simulink model "fi_at"  (R2026a)
settings: Solver=ode5  StopTime=30  FixedStep=.01  AbsTol=1e-6
model workspace (MATLAB code in the model file):
  | load sldemo_autotrans_data; %load initial conditions and other necessary data
undefined symbols (not defined in the file or in its folder): converter_data, downtab, emap, Iei, uptab, vehicledata
Description:
  | Modeling an Automatic Transmission Controller
  | 
  | In this example, Simulink(R) is used to model an automotive drivetrain. Stateflow(R)
  | enhances the Simulink model with its representation of the transmission
  | control logic. Simulink provides a powerful environment for the modeling and
  | simulation of dynamic systems and processes. In many systems, though,
  | supervisory functions like changing modes or invoking new gain schedules must
  | respond to events that may occur and conditions that develop over time. As a
  | result, the environment requires a language capable of managing these multiple
  | modes and developing conditions. In the following example, Stateflow
  | demonstrates its strength in this capacity by performing the function of gear
  | selection in an automatic transmission. This function is combined with the
  | drivetrain dynamics in a natural and intuitive manner by incorporating a
  | Stateflow block in the Simulink block diagram.
settings Model: DataTypeOverride=Double  MinMaxOverflowLogging=ForceOff  SimulationMode=accelerator  ExtModeTrigMode=oneshot  ExtModeArmWhenConnect=off  ExtModeAutoUpdateStatusClock=off  Creator=The MathWorks Inc.  LastModifiedBy=harry_31916
settings DataIOCC: ExternalInput=[t__, u__]  SignalLoggingName=sldemo_autotrans_output
settings OptimizationCC: BooleanDataType=off  InitFltsAndDblsToZero=on
settings DebuggingCC: SaveWithParameterizedLinksMsg=none  UnderspecifiedInitializationDetection=Classic  CheckExecutionContextPreStartOutputMsg=on  SignalResolutionControl=TryResolveAllWithWarning  MultiTaskDSMMsg=warning  MultiTaskCondExecSysMsg=none  SigSpecEnsureSampleTimeMsg=none  IntegerOverflowMsg=none  IntegerSaturationMsg=none
settings HardwareCC: ProdHWDeviceType=32-bit Generic
settings SFSimCC: SFSimEcho=off
settings GRTTargetCC: TargetFcnLib=ansi_tfl_tmw.mat  CombineOutputUpdateFcns=off  GRTInterface=on
settings ConfigComp: CovMetricSettings=dcmtr

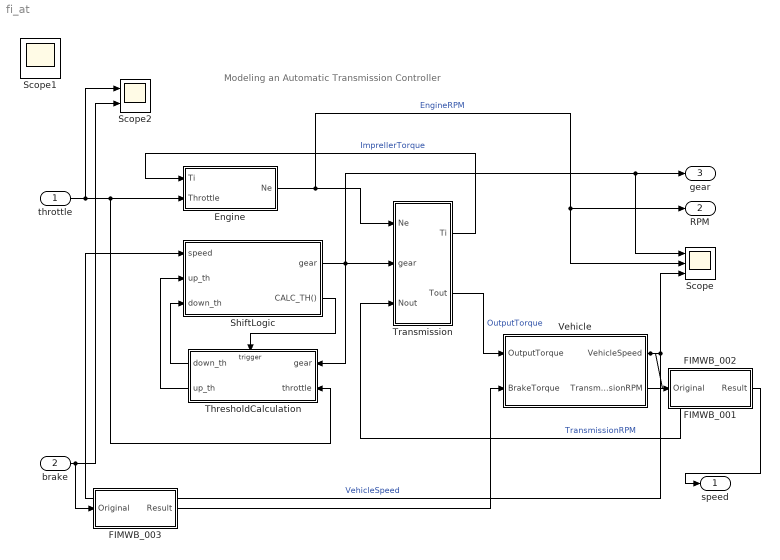
== system fi_at ==
  note: Modeling an Automatic Transmission Controller
  throttle : Inport  Interpolate=off
  brake : Inport  Port=2  Interpolate=off
  Engine : Subsystem
  FIMWB_001 : Subsystem  Tag=fimwb.fault.1
  FIMWB_002 : Subsystem  Tag=fimwb.fault.2
  FIMWB_003 : Subsystem  Tag=fimwb.fault.3
  Scope : Scope  NumInputPorts=3
      settings: ActiveDisplayYMinimum=-5  ActiveDisplayYMaximum=5
  Scope2 : Scope  NumInputPorts=2
      settings: ActiveDisplayYMinimum=-5  ActiveDisplayYMaximum=100
  ShiftLogic : Stateflow chart  TreatAsAtomicUnit=on
  ThresholdCalculation : Subsystem  TreatAsAtomicUnit=on
  Transmission : Subsystem
  Vehicle : Subsystem  mask(vehicle model){Rfd=vehicledata(1), rload0=vehicledata(2), rload2=vehicledata(3), Rw=vehicledata(4), Iv=vehicledata(5), N20=vehicledata(6)/vehicledata(4)*vehicledata(1)}
      mask prompts: Rfd "final drive ratio"; rload0 "drag friction at wheels"; rload2 "aerodynamic drag"; Rw "wheel radius"; Iv "vehicle inertia"; N20 "initial transmission output speed"
      mask help: vehicle dynamics: torque input from trans., outputs are input speed (transmission output) and vehicle speed
      mask Display: image(imread([matlabroot,'/toolbox/simulink/simdemos/automotive/html/NSX_3Colors.jpg']))
  speed : Outport  VectorParamsAs1DForOutWhenUnconnected=off
  RPM : Outport  Port=2  VectorParamsAs1DForOutWhenUnconnected=off
  gear : Outport  Port=3  VectorParamsAs1DForOutWhenUnconnected=off
  Scope1 : Scope
      settings: TimeSpan=30  ActiveDisplayYMinimum=1000  ActiveDisplayYMaximum=5000  DataLoggingMaxPoints=7500  DataLoggingSaveFormat=Array
  wires:
  Transmission/1(Ti) -> Engine/1(Ti)  "ImprellerTorque"
  Engine/1(Ne) -> Transmission/1(Ne), RPM/1, Scope/2  "EngineRPM"
  Vehicle/2(TransmissionRPM) -> Transmission/3(Nout)  "TransmissionRPM"
  ThresholdCalculation/1(down_th) -> ShiftLogic/3(down_th)
  ThresholdCalculation/2(up_th) -> ShiftLogic/2(up_th)
  ShiftLogic/1(gear) -> Transmission/2(gear), ThresholdCalculation/1(gear), gear/1, Scope/1
  ShiftLogic/2(CALC_TH()) -> ThresholdCalculation/Trigger
  Vehicle/1(VehicleSpeed) -> Scope/3, ShiftLogic/1(speed), FIMWB_001/1(Original)  "VehicleSpeed"
  throttle/1 -> Engine/2(Throttle), ThresholdCalculation/2(throttle), Scope2/1
  Transmission/2(Tout) -> Vehicle/1(OutputTorque)  "OutputTorque"
  brake/1 -> Scope2/2, FIMWB_003/1(Original)
  FIMWB_001/1(Result) -> FIMWB_002/1(Original)
  FIMWB_002/1(Result) -> speed/1
  FIMWB_003/1(Result) -> Vehicle/2(BrakeTorque)

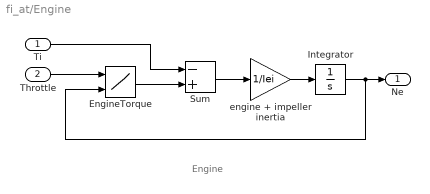
== system fi_at/Engine ==
  note: Engine
  Ti : Inport
  Throttle : Inport  Port=2
  EngineTorque : Lookup2D  RowIndex=thvec  ColumnIndex=nevec  Table=emap  SaturateOnIntegerOverflow=off
  Integrator : Integrator  InitialCondition=1000  LimitOutput=on  UpperSaturationLimit=6000  LowerSaturationLimit=600  ZeroCross=off
  Sum : Sum  Inputs=-+  InputSameDT=on  SaturateOnIntegerOverflow=on  OutDataTypeStr=Inherit: Same as first input
  engine + impeller inertia : Gain  Gain=1/Iei  SaturateOnIntegerOverflow=on  OutDataTypeStr=Inherit: Same as input  ParamDataTypeStr=Inherit: Same as input
  Ne : Outport  InitialOutput=0  VectorParamsAs1DForOutWhenUnconnected=off
  wires:
  Ti/1 -> Sum/1
  Throttle/1 -> EngineTorque/1
  Integrator/1 -> EngineTorque/2, Ne/1
  Sum/1 -> engine + impeller inertia/1
  engine + impeller inertia/1 -> Integrator/1
  EngineTorque/1 -> Sum/2

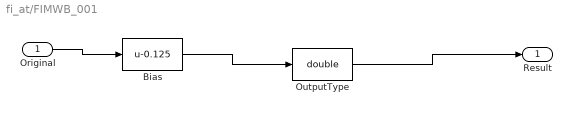
== system fi_at/FIMWB_001 ==
  Original : Inport
  Bias : Bias  Bias=-0.125  SaturateOnIntegerOverflow=off
  OutputType : DataTypeConversion  OutDataTypeStr=double  RndMeth=Round
  Result : Outport
  wires:
  Original/1 -> Bias/1
  Bias/1 -> OutputType/1
  OutputType/1 -> Result/1

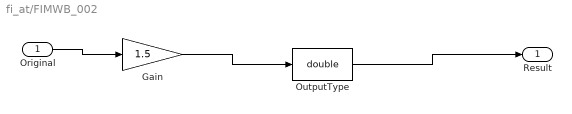
== system fi_at/FIMWB_002 ==
  Original : Inport
  Gain : Gain  Gain=1.5  OutDataTypeStr=Inherit: Same as input
  OutputType : DataTypeConversion  OutDataTypeStr=double  RndMeth=Round
  Result : Outport
  wires:
  Original/1 -> Gain/1
  Gain/1 -> OutputType/1
  OutputType/1 -> Result/1

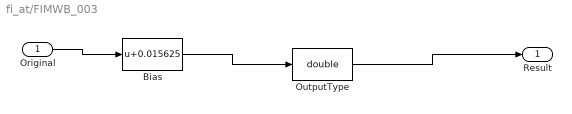
== system fi_at/FIMWB_003 ==
  Original : Inport
  Bias : Bias  Bias=0.015625  SaturateOnIntegerOverflow=off
  OutputType : DataTypeConversion  OutDataTypeStr=double  RndMeth=Round
  Result : Outport
  wires:
  Original/1 -> Bias/1
  Bias/1 -> OutputType/1
  OutputType/1 -> Result/1

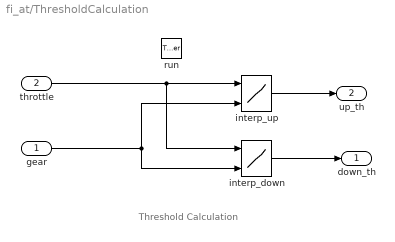
== system fi_at/ThresholdCalculation ==
  note: Threshold Calculation
  gear : Inport
  throttle : Inport  Port=2
  run : TriggerPort  TriggerType=function-call  VariantControl=(inherit)  ZeroCross=off
  interp_down : Lookup2D  RowIndex=downth  ColumnIndex=[1:4]  Table=downtab  OutDataTypeStr=double  SaturateOnIntegerOverflow=off  InputSameDT=off
      settings: LockScale=on
  interp_up : Lookup2D  RowIndex=upth  ColumnIndex=[1:4]  Table=uptab  OutDataTypeStr=double  SaturateOnIntegerOverflow=off  InputSameDT=off
      settings: LockScale=on
  down_th : Outport  VectorParamsAs1DForOutWhenUnconnected=off
  up_th : Outport  Port=2  VectorParamsAs1DForOutWhenUnconnected=off
  wires:
  interp_up/1 -> up_th/1
  interp_down/1 -> down_th/1
  throttle/1 -> interp_up/1, interp_down/1
  gear/1 -> interp_up/2, interp_down/2

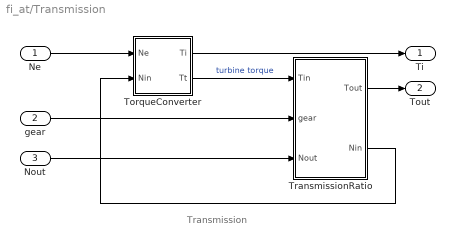
== system fi_at/Transmission ==
  note: Transmission
  Ne : Inport
  gear : Inport  Port=2
  Nout : Inport  Port=3
  TorqueConverter : Subsystem  mask(torque converter){speedratio=converter_data(:,1), Kfactor=converter_data(:,2), Torkratio=converter_data(:,3)}
      mask prompts: speedratio "speed ratio"; Kfactor "K factor"; Torkratio "torque ratio"
      mask help: torque converter
      mask Help: Torque converter input and output torques are computed as a function of the input and output speeds
      mask Display: plot([cos([90:10:450]*pi/180),.63*cos([90:10:450]*pi/180),.63*cos([90:10:240]*pi/180),cos([240:10:300]*pi/180),.63*cos([300]*pi/180)],[sin([90:10:450]*pi/180),.63*sin([90:10:450]*pi/180)+.1,.63*sin([90:10:240]*pi/180)+.1,sin([240:10:300]*pi/180),.63*sin([300]*pi/180)+.1])
  TransmissionRatio : Subsystem
  Ti : Outport  InitialOutput=0  VectorParamsAs1DForOutWhenUnconnected=off
  Tout : Outport  Port=2  InitialOutput=0  VectorParamsAs1DForOutWhenUnconnected=off
  wires:
  TransmissionRatio/1(Tout) -> Tout/1
  TorqueConverter/1(Ti) -> Ti/1
  Nout/1 -> TransmissionRatio/3(Nout)
  gear/1 -> TransmissionRatio/2(gear)
  Ne/1 -> TorqueConverter/1(Ne)
  TransmissionRatio/2(Nin) -> TorqueConverter/2(Nin)
  TorqueConverter/2(Tt) -> TransmissionRatio/1(Tin)  "turbine torque"

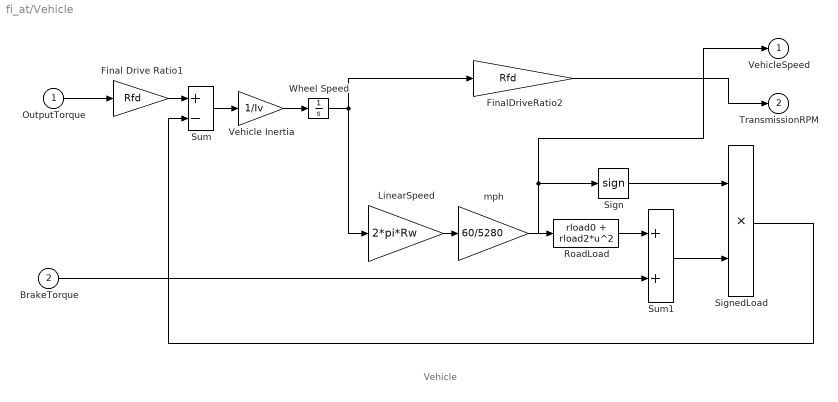
== system fi_at/Vehicle ==
  note: Vehicle
  OutputTorque : Inport
  BrakeTorque : Inport  Port=2
  Final Drive Ratio1 : Gain  Gain=Rfd  SaturateOnIntegerOverflow=on  OutDataTypeStr=Inherit: Same as input  ParamDataTypeStr=Inherit: Same as input
  FinalDriveRatio2 : Gain  Gain=Rfd  SaturateOnIntegerOverflow=on  OutDataTypeStr=Inherit: Same as input  ParamDataTypeStr=Inherit: Same as input
  LinearSpeed : Gain  Gain=2*pi*Rw  SaturateOnIntegerOverflow=on  OutDataTypeStr=Inherit: Same as input  ParamDataTypeStr=Inherit: Same as input
  RoadLoad : Fcn  Expr=rload0 + rload2*u^2
  Sign : Signum
  SignedLoad : Product  InputSameDT=on  SaturateOnIntegerOverflow=on  OutDataTypeStr=Inherit: Same as first input
  Sum : Sum  Inputs=+-  InputSameDT=on  SaturateOnIntegerOverflow=on  OutDataTypeStr=Inherit: Same as first input
  Sum1 : Sum  InputSameDT=on  SaturateOnIntegerOverflow=on  OutDataTypeStr=Inherit: Same as first input
  Vehicle Inertia : Gain  Gain=1/Iv  SaturateOnIntegerOverflow=on  OutDataTypeStr=Inherit: Same as input  ParamDataTypeStr=Inherit: Same as input
  Wheel Speed : Integrator  InitialCondition=N20/Rfd  ZeroCross=off
  mph : Gain  Gain=60/5280  SaturateOnIntegerOverflow=on  OutDataTypeStr=Inherit: Same as input  ParamDataTypeStr=Inherit: Same as input
  VehicleSpeed : Outport  InitialOutput=0  VectorParamsAs1DForOutWhenUnconnected=off
  TransmissionRPM : Outport  Port=2  InitialOutput=0  VectorParamsAs1DForOutWhenUnconnected=off
  wires:
  FinalDriveRatio2/1 -> TransmissionRPM/1
  BrakeTorque/1 -> Sum1/2
  Sum1/1 -> SignedLoad/2
  RoadLoad/1 -> Sum1/1
  Sign/1 -> SignedLoad/1
  SignedLoad/1 -> Sum/2
  OutputTorque/1 -> Final Drive Ratio1/1
  Vehicle Inertia/1 -> Wheel Speed/1
  Sum/1 -> Vehicle Inertia/1
  mph/1 -> VehicleSpeed/1, Sign/1, RoadLoad/1
  LinearSpeed/1 -> mph/1
  Wheel Speed/1 -> LinearSpeed/1, FinalDriveRatio2/1
  Final Drive Ratio1/1 -> Sum/1

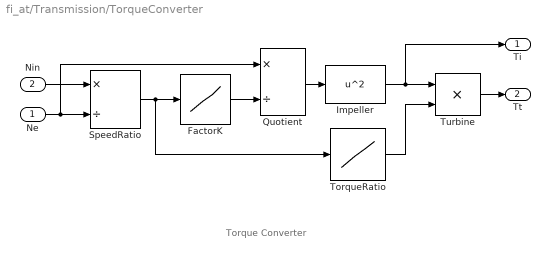
== system fi_at/Transmission/TorqueConverter ==
  note: Torque Converter
  Ne : Inport
  Nin : Inport  Port=2
  FactorK : Lookup  InputValues=speedratio  Table=Kfactor
  Impeller : Fcn  Expr=u^2
  Quotient : Product  Inputs=*/  InputSameDT=on  SaturateOnIntegerOverflow=on  OutDataTypeStr=Inherit: Same as first input
  SpeedRatio : Product  Inputs=*/  InputSameDT=on  SaturateOnIntegerOverflow=on  OutDataTypeStr=Inherit: Same as first input
  TorqueRatio : Lookup  InputValues=speedratio  Table=Torkratio
  Turbine : Product  InputSameDT=on  SaturateOnIntegerOverflow=on  OutDataTypeStr=Inherit: Same as first input
  Ti : Outport  InitialOutput=0  VectorParamsAs1DForOutWhenUnconnected=off
  Tt : Outport  Port=2  InitialOutput=0  VectorParamsAs1DForOutWhenUnconnected=off
  wires:
  TorqueRatio/1 -> Turbine/2
  Quotient/1 -> Impeller/1
  FactorK/1 -> Quotient/2
  SpeedRatio/1 -> TorqueRatio/1, FactorK/1
  Impeller/1 -> Turbine/1, Ti/1
  Turbine/1 -> Tt/1
  Ne/1 -> SpeedRatio/2, Quotient/1
  Nin/1 -> SpeedRatio/1

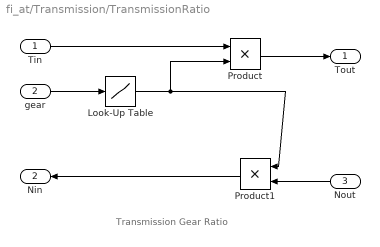
== system fi_at/Transmission/TransmissionRatio ==
  note: Transmission Gear Ratio
  Tin : Inport
  gear : Inport  Port=2
  Nout : Inport  Port=3
  Look-Up Table : Lookup  InputValues=[1 2 3 4]  Table=[2.393 1.450 1.000 0.677]  OutDataTypeStr=double  LockScale=on
  Product : Product  InputSameDT=on  SaturateOnIntegerOverflow=on  OutDataTypeStr=Inherit: Same as first input
  Product1 : Product  InputSameDT=on  SaturateOnIntegerOverflow=on  OutDataTypeStr=Inherit: Same as first input
  Tout : Outport  InitialOutput=0  VectorParamsAs1DForOutWhenUnconnected=off
  Nin : Outport  Port=2  InitialOutput=0  VectorParamsAs1DForOutWhenUnconnected=off
  wires:
  Look-Up Table/1 -> Product1/1, Product/2
  Nout/1 -> Product1/2
  Product1/1 -> Nin/1
  Product/1 -> Tout/1
  Tin/1 -> Product/1
  gear/1 -> Look-Up Table/1

== stateflow chart fi_at/ShiftLogic ==
  settings: updateMethod=DISCRETE  sampleTime=0.04
  state gear_state [parallel]
    settings: executionOrder=1
    state fourth
      entry:
      gear = 4;
    state third
      entry:
      gear = 3;
    state second
      entry:
      gear = 2;
    state first
      entry:
      gear = 1;
    (default) -> first
    second -> third [order 1] : UP
    first -> second : UP
    third -> fourth [order 1] : UP
    second -> first [order 2] : DOWN
    fourth -> third : DOWN
    third -> second [order 2] : DOWN
  state selection_state [parallel]
    during: CALC_TH;
    settings: executionOrder=2
    state steady_state
    state upshifting
    state downshifting
    (default) -> steady_state
    steady_state -> upshifting [order 1] : [speed > up_th]
    steady_state -> downshifting [order 2] : [speed < down_th]
    downshifting -> steady_state [order 1] : after(TWAIT,tick)
        | [speed <= down_th]
        | {gear_state.DOWN}
    downshifting -> steady_state [order 2] : [speed > down_th]
    upshifting -> steady_state [order 1] : after(TWAIT,tick)
        | [speed >= up_th]
        | {gear_state.UP}
    upshifting -> steady_state [order 2] : [speed < up_th]
  data: speed input double; gear output fixdt(0,8,5) [1..4]; TWAIT parameter fixdt(0,8,6); up_th input double; down_th input double
  events: DOWN local EITHER_EDGE_EVENT; UP local EITHER_EDGE_EVENT; CALC_TH output FUNCTION_CALL_EVENT
